simulink model "ASM_Traffic_new"  (R2024a)
settings: Solver=ode1  StartTime=SIM.tstart.v  StopTime=SIM.tend.v  FixedStep=SIM.StepSize.v  RelTol=1e-3
PostLoadFcn:
  | if any(exist('dsrtsu_mdlpostloadfcn', 'file') ~= 0), dsrtsu_mdlpostloadfcn('Execute', bdroot); end
  | try, asm_mdl_postloadfcn(bdroot, 'UpdateModel', 3600); catch, disp(lasterr); end,
InitFcn:
  | , if any(exist('rtifpga_mdlclblib', 'file') ~= 0), rtifpga_mdlclblib('Init', bdroot); end,
  | , if any(exist('dsmpb_private', 'file') ~= 0), dsmpb_private('dsmpb_mdlclblib', 'Init', bdroot); end,
undefined symbols (not defined in the file): _to_, a0b2, ASM_BrakeHydraulics_DemoSystems, ASM_VehicleDynamics_DemoSystems, b98103fe8ad365046cd0, BrakeCircuit, CPT, Crankshaft, DiscIntNeverNeededParam, dsmsi, FinalDriveAssembly, MDL, ModeSignals, Pos_BrakePedal_Maneuver, rad, RefSignals, s_to_rpm, SIM, SoftECU, Suspension, Tire, Transmission
libraries: ASM_Traffic_lib x135, simulink x100, ASM_Utils_lib x77, ASM_VehicleDynamics_lib x70, ASM_Environment_lib x22, dsmpblib x20, dsmsilib x15, MDLD_Utils_lib x10, ASM_BrakeHydraulics_lib x3
(part 61 of 63)

== system ASM_Traffic_new/Environment/GroundTruth/UserInterface/PAR_Plant/Fellow_Vehicles/Lightstates_Fellow25/Indicator_State[]/ASM_OSI_Mapping ==
  Fellow_TurnLights[] : Inport
  Table_ASM_To_OSI : Lookup_n-D  NumberOfTableDimensions=1  BreakpointsForDimension1=[0,1,2,3]  Table=[2,3,4,5]  InterpMethod=Nearest  InternalRulePriority=Speed  RndMeth=Simplest
  Indicator_State[] : Outport  VectorParamsAs1DForOutWhenUnconnected=off
  wires:
  Table_ASM_To_OSI/1 -> Indicator_State[]/1
  Fellow_TurnLights[]/1 -> Table_ASM_To_OSI/1

== system ASM_Traffic_new/Environment/GroundTruth/UserInterface/PAR_Plant/Fellow_Vehicles/Lightstates_Fellow26/Indicator_State[]/ASM_OSI_Mapping ==
  Fellow_TurnLights[] : Inport
  Table_ASM_To_OSI : Lookup_n-D  NumberOfTableDimensions=1  BreakpointsForDimension1=[0,1,2,3]  Table=[2,3,4,5]  InterpMethod=Nearest  InternalRulePriority=Speed  RndMeth=Simplest
  Indicator_State[] : Outport  VectorParamsAs1DForOutWhenUnconnected=off
  wires:
  Fellow_TurnLights[]/1 -> Table_ASM_To_OSI/1
  Table_ASM_To_OSI/1 -> Indicator_State[]/1

== system ASM_Traffic_new/Environment/GroundTruth/UserInterface/PAR_Plant/Fellow_Vehicles/Lightstates_Fellow27/Indicator_State[]/ASM_OSI_Mapping ==
  Fellow_TurnLights[] : Inport
  Table_ASM_To_OSI : Lookup_n-D  NumberOfTableDimensions=1  BreakpointsForDimension1=[0,1,2,3]  Table=[2,3,4,5]  InterpMethod=Nearest  InternalRulePriority=Speed  RndMeth=Simplest
  Indicator_State[] : Outport  VectorParamsAs1DForOutWhenUnconnected=off
  wires:
  Table_ASM_To_OSI/1 -> Indicator_State[]/1
  Fellow_TurnLights[]/1 -> Table_ASM_To_OSI/1

== system ASM_Traffic_new/Environment/GroundTruth/UserInterface/PAR_Plant/Fellow_Vehicles/Lightstates_Fellow28/Indicator_State[]/ASM_OSI_Mapping ==
  Fellow_TurnLights[] : Inport
  Table_ASM_To_OSI : Lookup_n-D  NumberOfTableDimensions=1  BreakpointsForDimension1=[0,1,2,3]  Table=[2,3,4,5]  InterpMethod=Nearest  InternalRulePriority=Speed  RndMeth=Simplest
  Indicator_State[] : Outport  VectorParamsAs1DForOutWhenUnconnected=off
  wires:
  Fellow_TurnLights[]/1 -> Table_ASM_To_OSI/1
  Table_ASM_To_OSI/1 -> Indicator_State[]/1

== system ASM_Traffic_new/Environment/GroundTruth/UserInterface/PAR_Plant/Fellow_Vehicles/Lightstates_Fellow29/Indicator_State[]/ASM_OSI_Mapping ==
  Fellow_TurnLights[] : Inport
  Table_ASM_To_OSI : Lookup_n-D  NumberOfTableDimensions=1  BreakpointsForDimension1=[0,1,2,3]  Table=[2,3,4,5]  InterpMethod=Nearest  InternalRulePriority=Speed  RndMeth=Simplest
  Indicator_State[] : Outport  VectorParamsAs1DForOutWhenUnconnected=off
  wires:
  Table_ASM_To_OSI/1 -> Indicator_State[]/1
  Fellow_TurnLights[]/1 -> Table_ASM_To_OSI/1

== system ASM_Traffic_new/Environment/GroundTruth/UserInterface/PAR_Plant/Fellow_Vehicles/Lightstates_Fellow3/Indicator_State[]/ASM_OSI_Mapping ==
  Fellow_TurnLights[] : Inport
  Table_ASM_To_OSI : Lookup_n-D  NumberOfTableDimensions=1  BreakpointsForDimension1=[0,1,2,3]  Table=[2,3,4,5]  InterpMethod=Nearest  InternalRulePriority=Speed  RndMeth=Simplest
  Indicator_State[] : Outport  VectorParamsAs1DForOutWhenUnconnected=off
  wires:
  Table_ASM_To_OSI/1 -> Indicator_State[]/1
  Fellow_TurnLights[]/1 -> Table_ASM_To_OSI/1

== system ASM_Traffic_new/Environment/GroundTruth/UserInterface/PAR_Plant/Fellow_Vehicles/Lightstates_Fellow30/Indicator_State[]/ASM_OSI_Mapping ==
  Fellow_TurnLights[] : Inport
  Table_ASM_To_OSI : Lookup_n-D  NumberOfTableDimensions=1  BreakpointsForDimension1=[0,1,2,3]  Table=[2,3,4,5]  InterpMethod=Nearest  InternalRulePriority=Speed  RndMeth=Simplest
  Indicator_State[] : Outport  VectorParamsAs1DForOutWhenUnconnected=off
  wires:
  Fellow_TurnLights[]/1 -> Table_ASM_To_OSI/1
  Table_ASM_To_OSI/1 -> Indicator_State[]/1

== system ASM_Traffic_new/Environment/GroundTruth/UserInterface/PAR_Plant/Fellow_Vehicles/Lightstates_Fellow4/Indicator_State[]/ASM_OSI_Mapping ==
  Fellow_TurnLights[] : Inport
  Table_ASM_To_OSI : Lookup_n-D  NumberOfTableDimensions=1  BreakpointsForDimension1=[0,1,2,3]  Table=[2,3,4,5]  InterpMethod=Nearest  InternalRulePriority=Speed  RndMeth=Simplest
  Indicator_State[] : Outport  VectorParamsAs1DForOutWhenUnconnected=off
  wires:
  Fellow_TurnLights[]/1 -> Table_ASM_To_OSI/1
  Table_ASM_To_OSI/1 -> Indicator_State[]/1

== system ASM_Traffic_new/Environment/GroundTruth/UserInterface/PAR_Plant/Fellow_Vehicles/Lightstates_Fellow5/Indicator_State[]/ASM_OSI_Mapping ==
  Fellow_TurnLights[] : Inport
  Table_ASM_To_OSI : Lookup_n-D  NumberOfTableDimensions=1  BreakpointsForDimension1=[0,1,2,3]  Table=[2,3,4,5]  InterpMethod=Nearest  InternalRulePriority=Speed  RndMeth=Simplest
  Indicator_State[] : Outport  VectorParamsAs1DForOutWhenUnconnected=off
  wires:
  Table_ASM_To_OSI/1 -> Indicator_State[]/1
  Fellow_TurnLights[]/1 -> Table_ASM_To_OSI/1

== system ASM_Traffic_new/Environment/GroundTruth/UserInterface/PAR_Plant/Fellow_Vehicles/Lightstates_Fellow6/Indicator_State[]/ASM_OSI_Mapping ==
  Fellow_TurnLights[] : Inport
  Table_ASM_To_OSI : Lookup_n-D  NumberOfTableDimensions=1  BreakpointsForDimension1=[0,1,2,3]  Table=[2,3,4,5]  InterpMethod=Nearest  InternalRulePriority=Speed  RndMeth=Simplest
  Indicator_State[] : Outport  VectorParamsAs1DForOutWhenUnconnected=off
  wires:
  Fellow_TurnLights[]/1 -> Table_ASM_To_OSI/1
  Table_ASM_To_OSI/1 -> Indicator_State[]/1

== system ASM_Traffic_new/Environment/GroundTruth/UserInterface/PAR_Plant/Fellow_Vehicles/Lightstates_Fellow7/Indicator_State[]/ASM_OSI_Mapping ==
  Fellow_TurnLights[] : Inport
  Table_ASM_To_OSI : Lookup_n-D  NumberOfTableDimensions=1  BreakpointsForDimension1=[0,1,2,3]  Table=[2,3,4,5]  InterpMethod=Nearest  InternalRulePriority=Speed  RndMeth=Simplest
  Indicator_State[] : Outport  VectorParamsAs1DForOutWhenUnconnected=off
  wires:
  Table_ASM_To_OSI/1 -> Indicator_State[]/1
  Fellow_TurnLights[]/1 -> Table_ASM_To_OSI/1

== system ASM_Traffic_new/Environment/GroundTruth/UserInterface/PAR_Plant/Fellow_Vehicles/Lightstates_Fellow8/Indicator_State[]/ASM_OSI_Mapping ==
  Fellow_TurnLights[] : Inport
  Table_ASM_To_OSI : Lookup_n-D  NumberOfTableDimensions=1  BreakpointsForDimension1=[0,1,2,3]  Table=[2,3,4,5]  InterpMethod=Nearest  InternalRulePriority=Speed  RndMeth=Simplest
  Indicator_State[] : Outport  VectorParamsAs1DForOutWhenUnconnected=off
  wires:
  Fellow_TurnLights[]/1 -> Table_ASM_To_OSI/1
  Table_ASM_To_OSI/1 -> Indicator_State[]/1

== system ASM_Traffic_new/Environment/GroundTruth/UserInterface/PAR_Plant/Fellow_Vehicles/Lightstates_Fellow9/Indicator_State[]/ASM_OSI_Mapping ==
  Fellow_TurnLights[] : Inport
  Table_ASM_To_OSI : Lookup_n-D  NumberOfTableDimensions=1  BreakpointsForDimension1=[0,1,2,3]  Table=[2,3,4,5]  InterpMethod=Nearest  InternalRulePriority=Speed  RndMeth=Simplest
  Indicator_State[] : Outport  VectorParamsAs1DForOutWhenUnconnected=off
  wires:
  Table_ASM_To_OSI/1 -> Indicator_State[]/1
  Fellow_TurnLights[]/1 -> Table_ASM_To_OSI/1

== system ASM_Traffic_new/Environment/Sensors/PlantModel/Object_Sensor_2D/ObjectData/Sensor1/Object_Custom_Values/Vectorize_Signals ==
  SensorOutput1 : Inport
  SensorOutput2 : Inport  Port=2
  SensorOutput3 : Inport  Port=3
  Bus Creator : BusCreator  Inputs=2
  Bus Selector : BusSelector  OutputSignals=SensorOutput.Object1.Object_Valid[0|1],SensorOutput.Object2.Object_Valid[0|1],SensorOutput.Object3.Object_Valid[0|1],SensorOutput.Object4.Object_Valid[0|1],SensorOutput.Object5.Object_Valid[0|1]
  Bus Selector1 : BusSelector  OutputSignals=SensorOutput.Object1.Object_Valid[0|1],SensorOutput.Object2.Object_Valid[0|1],SensorOutput.Object3.Object_Valid[0|1],SensorOutput.Object4.Object_Valid[0|1],SensorOutput.Object5.Object_Valid[0|1]
  Bus Selector2 : BusSelector  OutputSignals=SensorOutput.Object1.Object_Valid[0|1],SensorOutput.Object2.Object_Valid[0|1],SensorOutput.Object3.Object_Valid[0|1],SensorOutput.Object4.Object_Valid[0|1],SensorOutput.Object5.Object_Valid[0|1]
  Bus Selector3 : BusSelector  OutputSignals=SensorOutput.Object1.CustomValues[],SensorOutput.Object2.CustomValues[],SensorOutput.Object3.CustomValues[],SensorOutput.Object4.CustomValues[],SensorOutput.Object5.CustomValues[]
  Bus Selector4 : BusSelector  OutputSignals=SensorOutput.Object1.CustomValues[],SensorOutput.Object2.CustomValues[],SensorOutput.Object3.CustomValues[],SensorOutput.Object4.CustomValues[],SensorOutput.Object5.CustomValues[]
  Bus Selector5 : BusSelector  OutputSignals=SensorOutput.Object1.CustomValues[],SensorOutput.Object2.CustomValues[],SensorOutput.Object3.CustomValues[],SensorOutput.Object4.CustomValues[],SensorOutput.Object5.CustomValues[]
  Mux : Mux  Inputs=15
  Mux1 : Mux  Inputs=15
  Vectorized_Custom_Values : Outport  VectorParamsAs1DForOutWhenUnconnected=off
  wires:
  Bus Creator/1 -> Vectorized_Custom_Values/1
  Bus Selector5/5 -> Mux1/15  "<CustomValues[]>"
  Bus Selector5/4 -> Mux1/14  "<CustomValues[]>"
  Bus Selector5/3 -> Mux1/13  "<CustomValues[]>"
  Bus Selector5/2 -> Mux1/12  "<CustomValues[]>"
  Bus Selector5/1 -> Mux1/11  "<CustomValues[]>"
  Bus Selector4/5 -> Mux1/10  "<CustomValues[]>"
  Bus Selector4/4 -> Mux1/9  "<CustomValues[]>"
  Bus Selector4/3 -> Mux1/8  "<CustomValues[]>"
  Bus Selector4/2 -> Mux1/7  "<CustomValues[]>"
  Bus Selector4/1 -> Mux1/6  "<CustomValues[]>"
  Bus Selector3/5 -> Mux1/5  "<CustomValues[]>"
  Bus Selector3/4 -> Mux1/4  "<CustomValues[]>"
  Bus Selector3/3 -> Mux1/3  "<CustomValues[]>"
  Bus Selector3/2 -> Mux1/2  "<CustomValues[]>"
  Bus Selector3/1 -> Mux1/1  "<CustomValues[]>"
  Bus Selector2/5 -> Mux/15  "<Object_Valid[0|1]>"
  Bus Selector2/4 -> Mux/14  "<Object_Valid[0|1]>"
  Bus Selector2/3 -> Mux/13  "<Object_Valid[0|1]>"
  Bus Selector2/2 -> Mux/12  "<Object_Valid[0|1]>"
  Bus Selector2/1 -> Mux/11  "<Object_Valid[0|1]>"
  Bus Selector1/5 -> Mux/10  "<Object_Valid[0|1]>"
  Bus Selector1/4 -> Mux/9  "<Object_Valid[0|1]>"
  Bus Selector1/3 -> Mux/8  "<Object_Valid[0|1]>"
  Bus Selector1/2 -> Mux/7  "<Object_Valid[0|1]>"
  Bus Selector1/1 -> Mux/6  "<Object_Valid[0|1]>"
  Mux1/1 -> Bus Creator/2  "CustomValues[]"
  Mux/1 -> Bus Creator/1  "Object_Valid[0|1]"
  SensorOutput3/1 -> Bus Selector2/1, Bus Selector5/1
  SensorOutput2/1 -> Bus Selector1/1, Bus Selector4/1
  Bus Selector/1 -> Mux/1  "<Object_Valid[0|1]>"
  Bus Selector/2 -> Mux/2  "<Object_Valid[0|1]>"
  Bus Selector/3 -> Mux/3  "<Object_Valid[0|1]>"
  Bus Selector/4 -> Mux/4  "<Object_Valid[0|1]>"
  Bus Selector/5 -> Mux/5  "<Object_Valid[0|1]>"
  SensorOutput1/1 -> Bus Selector3/1, Bus Selector/1

== system ASM_Traffic_new/Environment/Sensors/PlantModel/Object_Sensor_2D/ObjectData/Sensor2/Object_Custom_Values/Vectorize_Signals ==
  SensorOutput1 : Inport
  SensorOutput2 : Inport  Port=2
  SensorOutput3 : Inport  Port=3
  Bus Creator : BusCreator  Inputs=2
  Bus Selector : BusSelector  OutputSignals=SensorOutput.Object1.Object_Valid[0|1],SensorOutput.Object2.Object_Valid[0|1],SensorOutput.Object3.Object_Valid[0|1],SensorOutput.Object4.Object_Valid[0|1],SensorOutput.Object5.Object_Valid[0|1]
  Bus Selector1 : BusSelector  OutputSignals=SensorOutput.Object1.Object_Valid[0|1],SensorOutput.Object2.Object_Valid[0|1],SensorOutput.Object3.Object_Valid[0|1],SensorOutput.Object4.Object_Valid[0|1],SensorOutput.Object5.Object_Valid[0|1]
  Bus Selector2 : BusSelector  OutputSignals=SensorOutput.Object1.Object_Valid[0|1],SensorOutput.Object2.Object_Valid[0|1],SensorOutput.Object3.Object_Valid[0|1],SensorOutput.Object4.Object_Valid[0|1],SensorOutput.Object5.Object_Valid[0|1]
  Bus Selector3 : BusSelector  OutputSignals=SensorOutput.Object1.CustomValues[],SensorOutput.Object2.CustomValues[],SensorOutput.Object3.CustomValues[],SensorOutput.Object4.CustomValues[],SensorOutput.Object5.CustomValues[]
  Bus Selector4 : BusSelector  OutputSignals=SensorOutput.Object1.CustomValues[],SensorOutput.Object2.CustomValues[],SensorOutput.Object3.CustomValues[],SensorOutput.Object4.CustomValues[],SensorOutput.Object5.CustomValues[]
  Bus Selector5 : BusSelector  OutputSignals=SensorOutput.Object1.CustomValues[],SensorOutput.Object2.CustomValues[],SensorOutput.Object3.CustomValues[],SensorOutput.Object4.CustomValues[],SensorOutput.Object5.CustomValues[]
  Mux : Mux  Inputs=15
  Mux1 : Mux  Inputs=15
  Vectorized_Custom_Values : Outport  VectorParamsAs1DForOutWhenUnconnected=off
  wires:
  SensorOutput1/1 -> Bus Selector/1, Bus Selector3/1
  Bus Selector/5 -> Mux/5  "<Object_Valid[0|1]>"
  Bus Selector/4 -> Mux/4  "<Object_Valid[0|1]>"
  Bus Selector/3 -> Mux/3  "<Object_Valid[0|1]>"
  Bus Selector/2 -> Mux/2  "<Object_Valid[0|1]>"
  Bus Selector/1 -> Mux/1  "<Object_Valid[0|1]>"
  SensorOutput2/1 -> Bus Selector4/1, Bus Selector1/1
  SensorOutput3/1 -> Bus Selector5/1, Bus Selector2/1
  Mux/1 -> Bus Creator/1  "Object_Valid[0|1]"
  Mux1/1 -> Bus Creator/2  "CustomValues[]"
  Bus Selector1/1 -> Mux/6  "<Object_Valid[0|1]>"
  Bus Selector1/2 -> Mux/7  "<Object_Valid[0|1]>"
  Bus Selector1/3 -> Mux/8  "<Object_Valid[0|1]>"
  Bus Selector1/4 -> Mux/9  "<Object_Valid[0|1]>"
  Bus Selector1/5 -> Mux/10  "<Object_Valid[0|1]>"
  Bus Selector2/1 -> Mux/11  "<Object_Valid[0|1]>"
  Bus Selector2/2 -> Mux/12  "<Object_Valid[0|1]>"
  Bus Selector2/3 -> Mux/13  "<Object_Valid[0|1]>"
  Bus Selector2/4 -> Mux/14  "<Object_Valid[0|1]>"
  Bus Selector2/5 -> Mux/15  "<Object_Valid[0|1]>"
  Bus Selector3/1 -> Mux1/1  "<CustomValues[]>"
  Bus Selector3/2 -> Mux1/2  "<CustomValues[]>"
  Bus Selector3/3 -> Mux1/3  "<CustomValues[]>"
  Bus Selector3/4 -> Mux1/4  "<CustomValues[]>"
  Bus Selector3/5 -> Mux1/5  "<CustomValues[]>"
  Bus Selector4/1 -> Mux1/6  "<CustomValues[]>"
  Bus Selector4/2 -> Mux1/7  "<CustomValues[]>"
  Bus Selector4/3 -> Mux1/8  "<CustomValues[]>"
  Bus Selector4/4 -> Mux1/9  "<CustomValues[]>"
  Bus Selector4/5 -> Mux1/10  "<CustomValues[]>"
  Bus Selector5/1 -> Mux1/11  "<CustomValues[]>"
  Bus Selector5/2 -> Mux1/12  "<CustomValues[]>"
  Bus Selector5/3 -> Mux1/13  "<CustomValues[]>"
  Bus Selector5/4 -> Mux1/14  "<CustomValues[]>"
  Bus Selector5/5 -> Mux1/15  "<CustomValues[]>"
  Bus Creator/1 -> Vectorized_Custom_Values/1

== system ASM_Traffic_new/Environment/Sensors/PlantModel/Object_Sensor_2D/ObjectData/Sensor3/Object_Custom_Values/Vectorize_Signals ==
  SensorOutput1 : Inport
  SensorOutput2 : Inport  Port=2
  SensorOutput3 : Inport  Port=3
  Bus Creator : BusCreator  Inputs=2
  Bus Selector : BusSelector  OutputSignals=SensorOutput.Object1.Object_Valid[0|1],SensorOutput.Object2.Object_Valid[0|1],SensorOutput.Object3.Object_Valid[0|1],SensorOutput.Object4.Object_Valid[0|1],SensorOutput.Object5.Object_Valid[0|1]
  Bus Selector1 : BusSelector  OutputSignals=SensorOutput.Object1.Object_Valid[0|1],SensorOutput.Object2.Object_Valid[0|1],SensorOutput.Object3.Object_Valid[0|1],SensorOutput.Object4.Object_Valid[0|1],SensorOutput.Object5.Object_Valid[0|1]
  Bus Selector2 : BusSelector  OutputSignals=SensorOutput.Object1.Object_Valid[0|1],SensorOutput.Object2.Object_Valid[0|1],SensorOutput.Object3.Object_Valid[0|1],SensorOutput.Object4.Object_Valid[0|1],SensorOutput.Object5.Object_Valid[0|1]
  Bus Selector3 : BusSelector  OutputSignals=SensorOutput.Object1.CustomValues[],SensorOutput.Object2.CustomValues[],SensorOutput.Object3.CustomValues[],SensorOutput.Object4.CustomValues[],SensorOutput.Object5.CustomValues[]
  Bus Selector4 : BusSelector  OutputSignals=SensorOutput.Object1.CustomValues[],SensorOutput.Object2.CustomValues[],SensorOutput.Object3.CustomValues[],SensorOutput.Object4.CustomValues[],SensorOutput.Object5.CustomValues[]
  Bus Selector5 : BusSelector  OutputSignals=SensorOutput.Object1.CustomValues[],SensorOutput.Object2.CustomValues[],SensorOutput.Object3.CustomValues[],SensorOutput.Object4.CustomValues[],SensorOutput.Object5.CustomValues[]
  Mux : Mux  Inputs=15
  Mux1 : Mux  Inputs=15
  Vectorized_Custom_Values : Outport  VectorParamsAs1DForOutWhenUnconnected=off
  wires:
  Bus Creator/1 -> Vectorized_Custom_Values/1
  Bus Selector5/5 -> Mux1/15  "<CustomValues[]>"
  Bus Selector5/4 -> Mux1/14  "<CustomValues[]>"
  Bus Selector5/3 -> Mux1/13  "<CustomValues[]>"
  Bus Selector5/2 -> Mux1/12  "<CustomValues[]>"
  Bus Selector5/1 -> Mux1/11  "<CustomValues[]>"
  Bus Selector4/5 -> Mux1/10  "<CustomValues[]>"
  Bus Selector4/4 -> Mux1/9  "<CustomValues[]>"
  Bus Selector4/3 -> Mux1/8  "<CustomValues[]>"
  Bus Selector4/2 -> Mux1/7  "<CustomValues[]>"
  Bus Selector4/1 -> Mux1/6  "<CustomValues[]>"
  Bus Selector3/5 -> Mux1/5  "<CustomValues[]>"
  Bus Selector3/4 -> Mux1/4  "<CustomValues[]>"
  Bus Selector3/3 -> Mux1/3  "<CustomValues[]>"
  Bus Selector3/2 -> Mux1/2  "<CustomValues[]>"
  Bus Selector3/1 -> Mux1/1  "<CustomValues[]>"
  Bus Selector2/5 -> Mux/15  "<Object_Valid[0|1]>"
  Bus Selector2/4 -> Mux/14  "<Object_Valid[0|1]>"
  Bus Selector2/3 -> Mux/13  "<Object_Valid[0|1]>"
  Bus Selector2/2 -> Mux/12  "<Object_Valid[0|1]>"
  Bus Selector2/1 -> Mux/11  "<Object_Valid[0|1]>"
  Bus Selector1/5 -> Mux/10  "<Object_Valid[0|1]>"
  Bus Selector1/4 -> Mux/9  "<Object_Valid[0|1]>"
  Bus Selector1/3 -> Mux/8  "<Object_Valid[0|1]>"
  Bus Selector1/2 -> Mux/7  "<Object_Valid[0|1]>"
  Bus Selector1/1 -> Mux/6  "<Object_Valid[0|1]>"
  Mux1/1 -> Bus Creator/2  "CustomValues[]"
  Mux/1 -> Bus Creator/1  "Object_Valid[0|1]"
  SensorOutput3/1 -> Bus Selector2/1, Bus Selector5/1
  SensorOutput2/1 -> Bus Selector1/1, Bus Selector4/1
  Bus Selector/1 -> Mux/1  "<Object_Valid[0|1]>"
  Bus Selector/2 -> Mux/2  "<Object_Valid[0|1]>"
  Bus Selector/3 -> Mux/3  "<Object_Valid[0|1]>"
  Bus Selector/4 -> Mux/4  "<Object_Valid[0|1]>"
  Bus Selector/5 -> Mux/5  "<Object_Valid[0|1]>"
  SensorOutput1/1 -> Bus Selector3/1, Bus Selector/1

== system ASM_Traffic_new/Environment/Sensors/PlantModel/Object_Sensor_2D/ObjectData/Sensor4/Object_Custom_Values/Vectorize_Signals ==
  SensorOutput1 : Inport
  SensorOutput2 : Inport  Port=2
  SensorOutput3 : Inport  Port=3
  Bus Creator : BusCreator  Inputs=2
  Bus Selector : BusSelector  OutputSignals=SensorOutput.Object1.Object_Valid[0|1],SensorOutput.Object2.Object_Valid[0|1],SensorOutput.Object3.Object_Valid[0|1],SensorOutput.Object4.Object_Valid[0|1],SensorOutput.Object5.Object_Valid[0|1]
  Bus Selector1 : BusSelector  OutputSignals=SensorOutput.Object1.Object_Valid[0|1],SensorOutput.Object2.Object_Valid[0|1],SensorOutput.Object3.Object_Valid[0|1],SensorOutput.Object4.Object_Valid[0|1],SensorOutput.Object5.Object_Valid[0|1]
  Bus Selector2 : BusSelector  OutputSignals=SensorOutput.Object1.Object_Valid[0|1],SensorOutput.Object2.Object_Valid[0|1],SensorOutput.Object3.Object_Valid[0|1],SensorOutput.Object4.Object_Valid[0|1],SensorOutput.Object5.Object_Valid[0|1]
  Bus Selector3 : BusSelector  OutputSignals=SensorOutput.Object1.CustomValues[],SensorOutput.Object2.CustomValues[],SensorOutput.Object3.CustomValues[],SensorOutput.Object4.CustomValues[],SensorOutput.Object5.CustomValues[]
  Bus Selector4 : BusSelector  OutputSignals=SensorOutput.Object1.CustomValues[],SensorOutput.Object2.CustomValues[],SensorOutput.Object3.CustomValues[],SensorOutput.Object4.CustomValues[],SensorOutput.Object5.CustomValues[]
  Bus Selector5 : BusSelector  OutputSignals=SensorOutput.Object1.CustomValues[],SensorOutput.Object2.CustomValues[],SensorOutput.Object3.CustomValues[],SensorOutput.Object4.CustomValues[],SensorOutput.Object5.CustomValues[]
  Mux : Mux  Inputs=15
  Mux1 : Mux  Inputs=15
  Vectorized_Custom_Values : Outport  VectorParamsAs1DForOutWhenUnconnected=off
  wires:
  Bus Creator/1 -> Vectorized_Custom_Values/1
  Bus Selector5/5 -> Mux1/15  "<CustomValues[]>"
  Bus Selector5/4 -> Mux1/14  "<CustomValues[]>"
  Bus Selector5/3 -> Mux1/13  "<CustomValues[]>"
  Bus Selector5/2 -> Mux1/12  "<CustomValues[]>"
  Bus Selector5/1 -> Mux1/11  "<CustomValues[]>"
  Bus Selector4/5 -> Mux1/10  "<CustomValues[]>"
  Bus Selector4/4 -> Mux1/9  "<CustomValues[]>"
  Bus Selector4/3 -> Mux1/8  "<CustomValues[]>"
  Bus Selector4/2 -> Mux1/7  "<CustomValues[]>"
  Bus Selector4/1 -> Mux1/6  "<CustomValues[]>"
  Bus Selector3/5 -> Mux1/5  "<CustomValues[]>"
  Bus Selector3/4 -> Mux1/4  "<CustomValues[]>"
  Bus Selector3/3 -> Mux1/3  "<CustomValues[]>"
  Bus Selector3/2 -> Mux1/2  "<CustomValues[]>"
  Bus Selector3/1 -> Mux1/1  "<CustomValues[]>"
  Bus Selector2/5 -> Mux/15  "<Object_Valid[0|1]>"
  Bus Selector2/4 -> Mux/14  "<Object_Valid[0|1]>"
  Bus Selector2/3 -> Mux/13  "<Object_Valid[0|1]>"
  Bus Selector2/2 -> Mux/12  "<Object_Valid[0|1]>"
  Bus Selector2/1 -> Mux/11  "<Object_Valid[0|1]>"
  Bus Selector1/5 -> Mux/10  "<Object_Valid[0|1]>"
  Bus Selector1/4 -> Mux/9  "<Object_Valid[0|1]>"
  Bus Selector1/3 -> Mux/8  "<Object_Valid[0|1]>"
  Bus Selector1/2 -> Mux/7  "<Object_Valid[0|1]>"
  Bus Selector1/1 -> Mux/6  "<Object_Valid[0|1]>"
  Mux1/1 -> Bus Creator/2  "CustomValues[]"
  Mux/1 -> Bus Creator/1  "Object_Valid[0|1]"
  SensorOutput3/1 -> Bus Selector2/1, Bus Selector5/1
  SensorOutput2/1 -> Bus Selector1/1, Bus Selector4/1
  Bus Selector/1 -> Mux/1  "<Object_Valid[0|1]>"
  Bus Selector/2 -> Mux/2  "<Object_Valid[0|1]>"
  Bus Selector/3 -> Mux/3  "<Object_Valid[0|1]>"
  Bus Selector/4 -> Mux/4  "<Object_Valid[0|1]>"
  Bus Selector/5 -> Mux/5  "<Object_Valid[0|1]>"
  SensorOutput1/1 -> Bus Selector3/1, Bus Selector/1

== system ASM_Traffic_new/Environment/Sensors/PlantModel/Object_Sensor_2D/ObjectData/Sensor5/Object_Custom_Values/Vectorize_Signals ==
  SensorOutput1 : Inport
  SensorOutput2 : Inport  Port=2
  SensorOutput3 : Inport  Port=3
  Bus Creator : BusCreator  Inputs=2
  Bus Selector : BusSelector  OutputSignals=SensorOutput.Object1.Object_Valid[0|1],SensorOutput.Object2.Object_Valid[0|1],SensorOutput.Object3.Object_Valid[0|1],SensorOutput.Object4.Object_Valid[0|1],SensorOutput.Object5.Object_Valid[0|1]
  Bus Selector1 : BusSelector  OutputSignals=SensorOutput.Object1.Object_Valid[0|1],SensorOutput.Object2.Object_Valid[0|1],SensorOutput.Object3.Object_Valid[0|1],SensorOutput.Object4.Object_Valid[0|1],SensorOutput.Object5.Object_Valid[0|1]
  Bus Selector2 : BusSelector  OutputSignals=SensorOutput.Object1.Object_Valid[0|1],SensorOutput.Object2.Object_Valid[0|1],SensorOutput.Object3.Object_Valid[0|1],SensorOutput.Object4.Object_Valid[0|1],SensorOutput.Object5.Object_Valid[0|1]
  Bus Selector3 : BusSelector  OutputSignals=SensorOutput.Object1.CustomValues[],SensorOutput.Object2.CustomValues[],SensorOutput.Object3.CustomValues[],SensorOutput.Object4.CustomValues[],SensorOutput.Object5.CustomValues[]
  Bus Selector4 : BusSelector  OutputSignals=SensorOutput.Object1.CustomValues[],SensorOutput.Object2.CustomValues[],SensorOutput.Object3.CustomValues[],SensorOutput.Object4.CustomValues[],SensorOutput.Object5.CustomValues[]
  Bus Selector5 : BusSelector  OutputSignals=SensorOutput.Object1.CustomValues[],SensorOutput.Object2.CustomValues[],SensorOutput.Object3.CustomValues[],SensorOutput.Object4.CustomValues[],SensorOutput.Object5.CustomValues[]
  Mux : Mux  Inputs=15
  Mux1 : Mux  Inputs=15
  Vectorized_Custom_Values : Outport  VectorParamsAs1DForOutWhenUnconnected=off
  wires:
  SensorOutput1/1 -> Bus Selector/1, Bus Selector3/1
  Bus Selector/5 -> Mux/5  "<Object_Valid[0|1]>"
  Bus Selector/4 -> Mux/4  "<Object_Valid[0|1]>"
  Bus Selector/3 -> Mux/3  "<Object_Valid[0|1]>"
  Bus Selector/2 -> Mux/2  "<Object_Valid[0|1]>"
  Bus Selector/1 -> Mux/1  "<Object_Valid[0|1]>"
  SensorOutput2/1 -> Bus Selector4/1, Bus Selector1/1
  SensorOutput3/1 -> Bus Selector5/1, Bus Selector2/1
  Mux/1 -> Bus Creator/1  "Object_Valid[0|1]"
  Mux1/1 -> Bus Creator/2  "CustomValues[]"
  Bus Selector1/1 -> Mux/6  "<Object_Valid[0|1]>"
  Bus Selector1/2 -> Mux/7  "<Object_Valid[0|1]>"
  Bus Selector1/3 -> Mux/8  "<Object_Valid[0|1]>"
  Bus Selector1/4 -> Mux/9  "<Object_Valid[0|1]>"
  Bus Selector1/5 -> Mux/10  "<Object_Valid[0|1]>"
  Bus Selector2/1 -> Mux/11  "<Object_Valid[0|1]>"
  Bus Selector2/2 -> Mux/12  "<Object_Valid[0|1]>"
  Bus Selector2/3 -> Mux/13  "<Object_Valid[0|1]>"
  Bus Selector2/4 -> Mux/14  "<Object_Valid[0|1]>"
  Bus Selector2/5 -> Mux/15  "<Object_Valid[0|1]>"
  Bus Selector3/1 -> Mux1/1  "<CustomValues[]>"
  Bus Selector3/2 -> Mux1/2  "<CustomValues[]>"
  Bus Selector3/3 -> Mux1/3  "<CustomValues[]>"
  Bus Selector3/4 -> Mux1/4  "<CustomValues[]>"
  Bus Selector3/5 -> Mux1/5  "<CustomValues[]>"
  Bus Selector4/1 -> Mux1/6  "<CustomValues[]>"
  Bus Selector4/2 -> Mux1/7  "<CustomValues[]>"
  Bus Selector4/3 -> Mux1/8  "<CustomValues[]>"
  Bus Selector4/4 -> Mux1/9  "<CustomValues[]>"
  Bus Selector4/5 -> Mux1/10  "<CustomValues[]>"
  Bus Selector5/1 -> Mux1/11  "<CustomValues[]>"
  Bus Selector5/2 -> Mux1/12  "<CustomValues[]>"
  Bus Selector5/3 -> Mux1/13  "<CustomValues[]>"
  Bus Selector5/4 -> Mux1/14  "<CustomValues[]>"
  Bus Selector5/5 -> Mux1/15  "<CustomValues[]>"
  Bus Creator/1 -> Vectorized_Custom_Values/1

== system ASM_Traffic_new/Environment/Sensors/PlantModel/Object_Sensor_2D/ObjectData/Sensor6/Object_Custom_Values/Vectorize_Signals ==
  SensorOutput1 : Inport
  SensorOutput2 : Inport  Port=2
  SensorOutput3 : Inport  Port=3
  Bus Creator : BusCreator  Inputs=2
  Bus Selector : BusSelector  OutputSignals=SensorOutput.Object1.Object_Valid[0|1],SensorOutput.Object2.Object_Valid[0|1],SensorOutput.Object3.Object_Valid[0|1],SensorOutput.Object4.Object_Valid[0|1],SensorOutput.Object5.Object_Valid[0|1]
  Bus Selector1 : BusSelector  OutputSignals=SensorOutput.Object1.Object_Valid[0|1],SensorOutput.Object2.Object_Valid[0|1],SensorOutput.Object3.Object_Valid[0|1],SensorOutput.Object4.Object_Valid[0|1],SensorOutput.Object5.Object_Valid[0|1]
  Bus Selector2 : BusSelector  OutputSignals=SensorOutput.Object1.Object_Valid[0|1],SensorOutput.Object2.Object_Valid[0|1],SensorOutput.Object3.Object_Valid[0|1],SensorOutput.Object4.Object_Valid[0|1],SensorOutput.Object5.Object_Valid[0|1]
  Bus Selector3 : BusSelector  OutputSignals=SensorOutput.Object1.CustomValues[],SensorOutput.Object2.CustomValues[],SensorOutput.Object3.CustomValues[],SensorOutput.Object4.CustomValues[],SensorOutput.Object5.CustomValues[]
  Bus Selector4 : BusSelector  OutputSignals=SensorOutput.Object1.CustomValues[],SensorOutput.Object2.CustomValues[],SensorOutput.Object3.CustomValues[],SensorOutput.Object4.CustomValues[],SensorOutput.Object5.CustomValues[]
  Bus Selector5 : BusSelector  OutputSignals=SensorOutput.Object1.CustomValues[],SensorOutput.Object2.CustomValues[],SensorOutput.Object3.CustomValues[],SensorOutput.Object4.CustomValues[],SensorOutput.Object5.CustomValues[]
  Mux : Mux  Inputs=15
  Mux1 : Mux  Inputs=15
  Vectorized_Custom_Values : Outport  VectorParamsAs1DForOutWhenUnconnected=off
  wires:
  Bus Creator/1 -> Vectorized_Custom_Values/1
  Bus Selector5/5 -> Mux1/15  "<CustomValues[]>"
  Bus Selector5/4 -> Mux1/14  "<CustomValues[]>"
  Bus Selector5/3 -> Mux1/13  "<CustomValues[]>"
  Bus Selector5/2 -> Mux1/12  "<CustomValues[]>"
  Bus Selector5/1 -> Mux1/11  "<CustomValues[]>"
  Bus Selector4/5 -> Mux1/10  "<CustomValues[]>"
  Bus Selector4/4 -> Mux1/9  "<CustomValues[]>"
  Bus Selector4/3 -> Mux1/8  "<CustomValues[]>"
  Bus Selector4/2 -> Mux1/7  "<CustomValues[]>"
  Bus Selector4/1 -> Mux1/6  "<CustomValues[]>"
  Bus Selector3/5 -> Mux1/5  "<CustomValues[]>"
  Bus Selector3/4 -> Mux1/4  "<CustomValues[]>"
  Bus Selector3/3 -> Mux1/3  "<CustomValues[]>"
  Bus Selector3/2 -> Mux1/2  "<CustomValues[]>"
  Bus Selector3/1 -> Mux1/1  "<CustomValues[]>"
  Bus Selector2/5 -> Mux/15  "<Object_Valid[0|1]>"
  Bus Selector2/4 -> Mux/14  "<Object_Valid[0|1]>"
  Bus Selector2/3 -> Mux/13  "<Object_Valid[0|1]>"
  Bus Selector2/2 -> Mux/12  "<Object_Valid[0|1]>"
  Bus Selector2/1 -> Mux/11  "<Object_Valid[0|1]>"
  Bus Selector1/5 -> Mux/10  "<Object_Valid[0|1]>"
  Bus Selector1/4 -> Mux/9  "<Object_Valid[0|1]>"
  Bus Selector1/3 -> Mux/8  "<Object_Valid[0|1]>"
  Bus Selector1/2 -> Mux/7  "<Object_Valid[0|1]>"
  Bus Selector1/1 -> Mux/6  "<Object_Valid[0|1]>"
  Mux1/1 -> Bus Creator/2  "CustomValues[]"
  Mux/1 -> Bus Creator/1  "Object_Valid[0|1]"
  SensorOutput3/1 -> Bus Selector2/1, Bus Selector5/1
  SensorOutput2/1 -> Bus Selector1/1, Bus Selector4/1
  Bus Selector/1 -> Mux/1  "<Object_Valid[0|1]>"
  Bus Selector/2 -> Mux/2  "<Object_Valid[0|1]>"
  Bus Selector/3 -> Mux/3  "<Object_Valid[0|1]>"
  Bus Selector/4 -> Mux/4  "<Object_Valid[0|1]>"
  Bus Selector/5 -> Mux/5  "<Object_Valid[0|1]>"
  SensorOutput1/1 -> Bus Selector3/1, Bus Selector/1

== system ASM_Traffic_new/Environment/Sensors/PlantModel/Object_Sensor_2D/ObjectData/Sensor7/Object_Custom_Values/Vectorize_Signals ==
  SensorOutput1 : Inport
  SensorOutput2 : Inport  Port=2
  SensorOutput3 : Inport  Port=3
  Bus Creator : BusCreator  Inputs=2
  Bus Selector : BusSelector  OutputSignals=SensorOutput.Object1.Object_Valid[0|1],SensorOutput.Object2.Object_Valid[0|1],SensorOutput.Object3.Object_Valid[0|1],SensorOutput.Object4.Object_Valid[0|1],SensorOutput.Object5.Object_Valid[0|1]
  Bus Selector1 : BusSelector  OutputSignals=SensorOutput.Object1.Object_Valid[0|1],SensorOutput.Object2.Object_Valid[0|1],SensorOutput.Object3.Object_Valid[0|1],SensorOutput.Object4.Object_Valid[0|1],SensorOutput.Object5.Object_Valid[0|1]
  Bus Selector2 : BusSelector  OutputSignals=SensorOutput.Object1.Object_Valid[0|1],SensorOutput.Object2.Object_Valid[0|1],SensorOutput.Object3.Object_Valid[0|1],SensorOutput.Object4.Object_Valid[0|1],SensorOutput.Object5.Object_Valid[0|1]
  Bus Selector3 : BusSelector  OutputSignals=SensorOutput.Object1.CustomValues[],SensorOutput.Object2.CustomValues[],SensorOutput.Object3.CustomValues[],SensorOutput.Object4.CustomValues[],SensorOutput.Object5.CustomValues[]
  Bus Selector4 : BusSelector  OutputSignals=SensorOutput.Object1.CustomValues[],SensorOutput.Object2.CustomValues[],SensorOutput.Object3.CustomValues[],SensorOutput.Object4.CustomValues[],SensorOutput.Object5.CustomValues[]
  Bus Selector5 : BusSelector  OutputSignals=SensorOutput.Object1.CustomValues[],SensorOutput.Object2.CustomValues[],SensorOutput.Object3.CustomValues[],SensorOutput.Object4.CustomValues[],SensorOutput.Object5.CustomValues[]
  Mux : Mux  Inputs=15
  Mux1 : Mux  Inputs=15
  Vectorized_Custom_Values : Outport  VectorParamsAs1DForOutWhenUnconnected=off
  wires:
  SensorOutput1/1 -> Bus Selector/1, Bus Selector3/1
  Bus Selector/5 -> Mux/5  "<Object_Valid[0|1]>"
  Bus Selector/4 -> Mux/4  "<Object_Valid[0|1]>"
  Bus Selector/3 -> Mux/3  "<Object_Valid[0|1]>"
  Bus Selector/2 -> Mux/2  "<Object_Valid[0|1]>"
  Bus Selector/1 -> Mux/1  "<Object_Valid[0|1]>"
  SensorOutput2/1 -> Bus Selector4/1, Bus Selector1/1
  SensorOutput3/1 -> Bus Selector5/1, Bus Selector2/1
  Mux/1 -> Bus Creator/1  "Object_Valid[0|1]"
  Mux1/1 -> Bus Creator/2  "CustomValues[]"
  Bus Selector1/1 -> Mux/6  "<Object_Valid[0|1]>"
  Bus Selector1/2 -> Mux/7  "<Object_Valid[0|1]>"
  Bus Selector1/3 -> Mux/8  "<Object_Valid[0|1]>"
  Bus Selector1/4 -> Mux/9  "<Object_Valid[0|1]>"
  Bus Selector1/5 -> Mux/10  "<Object_Valid[0|1]>"
  Bus Selector2/1 -> Mux/11  "<Object_Valid[0|1]>"
  Bus Selector2/2 -> Mux/12  "<Object_Valid[0|1]>"
  Bus Selector2/3 -> Mux/13  "<Object_Valid[0|1]>"
  Bus Selector2/4 -> Mux/14  "<Object_Valid[0|1]>"
  Bus Selector2/5 -> Mux/15  "<Object_Valid[0|1]>"
  Bus Selector3/1 -> Mux1/1  "<CustomValues[]>"
  Bus Selector3/2 -> Mux1/2  "<CustomValues[]>"
  Bus Selector3/3 -> Mux1/3  "<CustomValues[]>"
  Bus Selector3/4 -> Mux1/4  "<CustomValues[]>"
  Bus Selector3/5 -> Mux1/5  "<CustomValues[]>"
  Bus Selector4/1 -> Mux1/6  "<CustomValues[]>"
  Bus Selector4/2 -> Mux1/7  "<CustomValues[]>"
  Bus Selector4/3 -> Mux1/8  "<CustomValues[]>"
  Bus Selector4/4 -> Mux1/9  "<CustomValues[]>"
  Bus Selector4/5 -> Mux1/10  "<CustomValues[]>"
  Bus Selector5/1 -> Mux1/11  "<CustomValues[]>"
  Bus Selector5/2 -> Mux1/12  "<CustomValues[]>"
  Bus Selector5/3 -> Mux1/13  "<CustomValues[]>"
  Bus Selector5/4 -> Mux1/14  "<CustomValues[]>"
  Bus Selector5/5 -> Mux1/15  "<CustomValues[]>"
  Bus Creator/1 -> Vectorized_Custom_Values/1

== system ASM_Traffic_new/Environment/Sensors/PlantModel/Object_Sensor_3D/CustomPoints/Sensor1/CustomPointsOutput/HoldSignals ==
  ResetPulse[0|1] : Inport
  CustomPoints_Signals_In[] : Inport  Port=2
  Enable : EnablePort
  Bus Selector1 : BusSelector  OutputSignals=Flag_In_Scope[0|1],Flag_Is_Occluded[0|1],ID[],Dist_CoorSys_S[m],v_CoorSys_S[m|s],v_CoorSys_S[x;y;z][m|s],a_CoorSys_S[m|s2],a_CoorSys_S[x;y;z][m|s2],Pos_CoorSys_S[x;y;z][m],Pos_CoorSys_E[x;y;z][m],Angle_Hor_CoorSys_S[deg],Angle_Ver_CoorSys_S[deg],Data_1[],Data_2[],Data_3[],Data_4[],Data_5[],Object_ID[],Object_Type[]
  CUSTOM_POINTS_SIGNALS_RESET_1 : ASM_Traffic_lib/Sensors/Custom Points/CUSTOM_POINTS_SIGNALS_RESET  ASMProperties=struct('Name','CUSTOM_POINTS_SIGNALS_RESET','Version','2.0','Library','ASM_Traffic_lib')  ASMInstanceName=custom_points_signals_reset  ASMInstanceID=1
  CustomPoints_Signals_Out[] : Outport  VectorParamsAs1DForOutWhenUnconnected=off
  wires:
  Bus Selector1/19 -> CUSTOM_POINTS_SIGNALS_RESET_1/20  "<Object_Type[]>"
  Bus Selector1/18 -> CUSTOM_POINTS_SIGNALS_RESET_1/19  "<Object_ID[]>"
  Bus Selector1/17 -> CUSTOM_POINTS_SIGNALS_RESET_1/18  "<Data_5[]>"
  Bus Selector1/16 -> CUSTOM_POINTS_SIGNALS_RESET_1/17  "<Data_4[]>"
  Bus Selector1/15 -> CUSTOM_POINTS_SIGNALS_RESET_1/16  "<Data_3[]>"
  Bus Selector1/14 -> CUSTOM_POINTS_SIGNALS_RESET_1/15  "<Data_2[]>"
  Bus Selector1/13 -> CUSTOM_POINTS_SIGNALS_RESET_1/14  "<Data_1[]>"
  Bus Selector1/12 -> CUSTOM_POINTS_SIGNALS_RESET_1/13  "<Angle_Ver_CoorSys_S[deg]>"
  Bus Selector1/11 -> CUSTOM_POINTS_SIGNALS_RESET_1/12  "<Angle_Hor_CoorSys_S[deg]>"
  Bus Selector1/10 -> CUSTOM_POINTS_SIGNALS_RESET_1/11  "<Pos_CoorSys_E[x;y;z][m]>"
  Bus Selector1/9 -> CUSTOM_POINTS_SIGNALS_RESET_1/10  "<Pos_CoorSys_S[x;y;z][m]>"
  Bus Selector1/8 -> CUSTOM_POINTS_SIGNALS_RESET_1/9  "<a_CoorSys_S[x;y;z][m|s2]>"
  Bus Selector1/7 -> CUSTOM_POINTS_SIGNALS_RESET_1/8  "<a_CoorSys_S[m|s2]>"
  Bus Selector1/6 -> CUSTOM_POINTS_SIGNALS_RESET_1/7  "<v_CoorSys_S[x;y;z][m|s]>"
  Bus Selector1/5 -> CUSTOM_POINTS_SIGNALS_RESET_1/6  "<v_CoorSys_S[m|s]>"
  Bus Selector1/4 -> CUSTOM_POINTS_SIGNALS_RESET_1/5  "<Dist_CoorSys_S[m]>"
  Bus Selector1/3 -> CUSTOM_POINTS_SIGNALS_RESET_1/4  "<ID[]>"
  Bus Selector1/2 -> CUSTOM_POINTS_SIGNALS_RESET_1/3  "<Flag_Is_Occluded[0|1]>"
  Bus Selector1/1 -> CUSTOM_POINTS_SIGNALS_RESET_1/2  "<Flag_In_Scope[0|1]>"
  CUSTOM_POINTS_SIGNALS_RESET_1/1 -> CustomPoints_Signals_Out[]/1
  ResetPulse[0|1]/1 -> CUSTOM_POINTS_SIGNALS_RESET_1/1
  CustomPoints_Signals_In[]/1 -> Bus Selector1/1

== system ASM_Traffic_new/Environment/Sensors/PlantModel/Object_Sensor_3D/CustomPoints/Sensor1/CustomPointsOutput/ResetPulse ==
  Enable[0|1] : Inport
  SensorActive[0|1] : Inport  Port=2
  Compare To Constant : simulink/Logic and Bit Operations/Compare To Constant  relop===  const=1  OutDataTypeStr=boolean
  Compare To Constant1 : simulink/Logic and Bit Operations/Compare To Constant  relop===  const=0  OutDataTypeStr=boolean
  Logical Operator1 : Logic  AllPortsSameDT=off  OutDataTypeStr=boolean
  Logical Operator2 : Logic  Operator=NAND  AllPortsSameDT=off  OutDataTypeStr=boolean
  Memory1 : UnitDelay  SampleTime=-1  HasFrameUpgradeWarning=on
  ResetPulse[0|1] : Outport  VectorParamsAs1DForOutWhenUnconnected=off
  wires:
  Enable[0|1]/1 -> Logical Operator2/2
  Compare To Constant1/1 -> Logical Operator1/2
  Compare To Constant/1 -> Logical Operator1/1
  Logical Operator1/1 -> ResetPulse[0|1]/1
  SensorActive[0|1]/1 -> Logical Operator2/1
  Logical Operator2/1 -> Memory1/1, Compare To Constant/1
  Memory1/1 -> Compare To Constant1/1

== system ASM_Traffic_new/Environment/Sensors/PlantModel/Object_Sensor_3D/CustomPoints/Sensor1/CustomPointsOutput/SignalBus ==
  CustomPoints_Signals_In[] : Inport
  Bus Creator : BusCreator  Inputs=5
  Bus Selector1 : BusSelector  OutputSignals=ID[],Object_ID[],Dist_CoorSys_S[m],Angle_Hor_CoorSys_S[deg],Pos_CoorSys_E[x;y;z][m]
  CustomPoints_Signals_Out[] : Outport  VectorParamsAs1DForOutWhenUnconnected=off
  wires:
  CustomPoints_Signals_In[]/1 -> Bus Selector1/1
  Bus Creator/1 -> CustomPoints_Signals_Out[]/1
  Bus Selector1/4 -> Bus Creator/4  "<Angle_Hor_CoorSys_S[deg]>"
  Bus Selector1/5 -> Bus Creator/5  "<Pos_CoorSys_E[x;y;z][m]>"
  Bus Selector1/2 -> Bus Creator/2  "<Object_ID[]>"
  Bus Selector1/3 -> Bus Creator/3  "<Dist_CoorSys_S[m]>"
  Bus Selector1/1 -> Bus Creator/1  "<ID[]>"

== system ASM_Traffic_new/Environment/Sensors/PlantModel/Object_Sensor_3D/CustomPoints/Sensor2/CustomPointsOutput/HoldSignals ==
  ResetPulse[0|1] : Inport
  CustomPoints_Signals_In[] : Inport  Port=2
  Enable : EnablePort
  Bus Selector1 : BusSelector  OutputSignals=Flag_In_Scope[0|1],Flag_Is_Occluded[0|1],ID[],Dist_CoorSys_S[m],v_CoorSys_S[m|s],v_CoorSys_S[x;y;z][m|s],a_CoorSys_S[m|s2],a_CoorSys_S[x;y;z][m|s2],Pos_CoorSys_S[x;y;z][m],Pos_CoorSys_E[x;y;z][m],Angle_Hor_CoorSys_S[deg],Angle_Ver_CoorSys_S[deg],Data_1[],Data_2[],Data_3[],Data_4[],Data_5[],Object_ID[],Object_Type[]
  CUSTOM_POINTS_SIGNALS_RESET_1 : ASM_Traffic_lib/Sensors/Custom Points/CUSTOM_POINTS_SIGNALS_RESET  ASMProperties=struct('Name','CUSTOM_POINTS_SIGNALS_RESET','Version','2.0','Library','ASM_Traffic_lib')  ASMInstanceName=custom_points_signals_reset  ASMInstanceID=1
  CustomPoints_Signals_Out[] : Outport  VectorParamsAs1DForOutWhenUnconnected=off
  wires:
  Bus Selector1/19 -> CUSTOM_POINTS_SIGNALS_RESET_1/20  "<Object_Type[]>"
  Bus Selector1/18 -> CUSTOM_POINTS_SIGNALS_RESET_1/19  "<Object_ID[]>"
  Bus Selector1/17 -> CUSTOM_POINTS_SIGNALS_RESET_1/18  "<Data_5[]>"
  Bus Selector1/16 -> CUSTOM_POINTS_SIGNALS_RESET_1/17  "<Data_4[]>"
  Bus Selector1/15 -> CUSTOM_POINTS_SIGNALS_RESET_1/16  "<Data_3[]>"
  Bus Selector1/14 -> CUSTOM_POINTS_SIGNALS_RESET_1/15  "<Data_2[]>"
  Bus Selector1/13 -> CUSTOM_POINTS_SIGNALS_RESET_1/14  "<Data_1[]>"
  Bus Selector1/12 -> CUSTOM_POINTS_SIGNALS_RESET_1/13  "<Angle_Ver_CoorSys_S[deg]>"
  Bus Selector1/11 -> CUSTOM_POINTS_SIGNALS_RESET_1/12  "<Angle_Hor_CoorSys_S[deg]>"
  Bus Selector1/10 -> CUSTOM_POINTS_SIGNALS_RESET_1/11  "<Pos_CoorSys_E[x;y;z][m]>"
  Bus Selector1/9 -> CUSTOM_POINTS_SIGNALS_RESET_1/10  "<Pos_CoorSys_S[x;y;z][m]>"
  Bus Selector1/8 -> CUSTOM_POINTS_SIGNALS_RESET_1/9  "<a_CoorSys_S[x;y;z][m|s2]>"
  Bus Selector1/7 -> CUSTOM_POINTS_SIGNALS_RESET_1/8  "<a_CoorSys_S[m|s2]>"
  Bus Selector1/6 -> CUSTOM_POINTS_SIGNALS_RESET_1/7  "<v_CoorSys_S[x;y;z][m|s]>"
  Bus Selector1/5 -> CUSTOM_POINTS_SIGNALS_RESET_1/6  "<v_CoorSys_S[m|s]>"
  Bus Selector1/4 -> CUSTOM_POINTS_SIGNALS_RESET_1/5  "<Dist_CoorSys_S[m]>"
  Bus Selector1/3 -> CUSTOM_POINTS_SIGNALS_RESET_1/4  "<ID[]>"
  Bus Selector1/2 -> CUSTOM_POINTS_SIGNALS_RESET_1/3  "<Flag_Is_Occluded[0|1]>"
  Bus Selector1/1 -> CUSTOM_POINTS_SIGNALS_RESET_1/2  "<Flag_In_Scope[0|1]>"
  CUSTOM_POINTS_SIGNALS_RESET_1/1 -> CustomPoints_Signals_Out[]/1
  ResetPulse[0|1]/1 -> CUSTOM_POINTS_SIGNALS_RESET_1/1
  CustomPoints_Signals_In[]/1 -> Bus Selector1/1

== system ASM_Traffic_new/Environment/Sensors/PlantModel/Object_Sensor_3D/CustomPoints/Sensor2/CustomPointsOutput/ResetPulse ==
  Enable[0|1] : Inport
  SensorActive[0|1] : Inport  Port=2
  Compare To Constant : simulink/Logic and Bit Operations/Compare To Constant  relop===  const=1  OutDataTypeStr=boolean
  Compare To Constant1 : simulink/Logic and Bit Operations/Compare To Constant  relop===  const=0  OutDataTypeStr=boolean
  Logical Operator1 : Logic  AllPortsSameDT=off  OutDataTypeStr=boolean
  Logical Operator2 : Logic  Operator=NAND  AllPortsSameDT=off  OutDataTypeStr=boolean
  Memory1 : UnitDelay  SampleTime=-1  HasFrameUpgradeWarning=on
  ResetPulse[0|1] : Outport  VectorParamsAs1DForOutWhenUnconnected=off
  wires:
  Enable[0|1]/1 -> Logical Operator2/2
  Compare To Constant1/1 -> Logical Operator1/2
  Compare To Constant/1 -> Logical Operator1/1
  Logical Operator1/1 -> ResetPulse[0|1]/1
  SensorActive[0|1]/1 -> Logical Operator2/1
  Logical Operator2/1 -> Memory1/1, Compare To Constant/1
  Memory1/1 -> Compare To Constant1/1

== system ASM_Traffic_new/Environment/Sensors/PlantModel/Object_Sensor_3D/CustomPoints/Sensor2/CustomPointsOutput/SignalBus ==
  CustomPoints_Signals_In[] : Inport
  Bus Creator : BusCreator  Inputs=5
  Bus Selector1 : BusSelector  OutputSignals=ID[],Object_ID[],Dist_CoorSys_S[m],Angle_Hor_CoorSys_S[deg],Pos_CoorSys_E[x;y;z][m]
  CustomPoints_Signals_Out[] : Outport  VectorParamsAs1DForOutWhenUnconnected=off
  wires:
  CustomPoints_Signals_In[]/1 -> Bus Selector1/1
  Bus Creator/1 -> CustomPoints_Signals_Out[]/1
  Bus Selector1/4 -> Bus Creator/4  "<Angle_Hor_CoorSys_S[deg]>"
  Bus Selector1/5 -> Bus Creator/5  "<Pos_CoorSys_E[x;y;z][m]>"
  Bus Selector1/2 -> Bus Creator/2  "<Object_ID[]>"
  Bus Selector1/3 -> Bus Creator/3  "<Dist_CoorSys_S[m]>"
  Bus Selector1/1 -> Bus Creator/1  "<ID[]>"

== system ASM_Traffic_new/Environment/Sensors/PlantModel/Object_Sensor_3D/CustomPoints/Sensor3/CustomPointsOutput/HoldSignals ==
  ResetPulse[0|1] : Inport
  CustomPoints_Signals_In[] : Inport  Port=2
  Enable : EnablePort
  Bus Selector1 : BusSelector  OutputSignals=Flag_In_Scope[0|1],Flag_Is_Occluded[0|1],ID[],Dist_CoorSys_S[m],v_CoorSys_S[m|s],v_CoorSys_S[x;y;z][m|s],a_CoorSys_S[m|s2],a_CoorSys_S[x;y;z][m|s2],Pos_CoorSys_S[x;y;z][m],Pos_CoorSys_E[x;y;z][m],Angle_Hor_CoorSys_S[deg],Angle_Ver_CoorSys_S[deg],Data_1[],Data_2[],Data_3[],Data_4[],Data_5[],Object_ID[],Object_Type[]
  CUSTOM_POINTS_SIGNALS_RESET_1 : ASM_Traffic_lib/Sensors/Custom Points/CUSTOM_POINTS_SIGNALS_RESET  ASMProperties=struct('Name','CUSTOM_POINTS_SIGNALS_RESET','Version','2.0','Library','ASM_Traffic_lib')  ASMInstanceName=custom_points_signals_reset  ASMInstanceID=1
  CustomPoints_Signals_Out[] : Outport  VectorParamsAs1DForOutWhenUnconnected=off
  wires:
  Bus Selector1/19 -> CUSTOM_POINTS_SIGNALS_RESET_1/20  "<Object_Type[]>"
  Bus Selector1/18 -> CUSTOM_POINTS_SIGNALS_RESET_1/19  "<Object_ID[]>"
  Bus Selector1/17 -> CUSTOM_POINTS_SIGNALS_RESET_1/18  "<Data_5[]>"
  Bus Selector1/16 -> CUSTOM_POINTS_SIGNALS_RESET_1/17  "<Data_4[]>"
  Bus Selector1/15 -> CUSTOM_POINTS_SIGNALS_RESET_1/16  "<Data_3[]>"
  Bus Selector1/14 -> CUSTOM_POINTS_SIGNALS_RESET_1/15  "<Data_2[]>"
  Bus Selector1/13 -> CUSTOM_POINTS_SIGNALS_RESET_1/14  "<Data_1[]>"
  Bus Selector1/12 -> CUSTOM_POINTS_SIGNALS_RESET_1/13  "<Angle_Ver_CoorSys_S[deg]>"
  Bus Selector1/11 -> CUSTOM_POINTS_SIGNALS_RESET_1/12  "<Angle_Hor_CoorSys_S[deg]>"
  Bus Selector1/10 -> CUSTOM_POINTS_SIGNALS_RESET_1/11  "<Pos_CoorSys_E[x;y;z][m]>"
  Bus Selector1/9 -> CUSTOM_POINTS_SIGNALS_RESET_1/10  "<Pos_CoorSys_S[x;y;z][m]>"
  Bus Selector1/8 -> CUSTOM_POINTS_SIGNALS_RESET_1/9  "<a_CoorSys_S[x;y;z][m|s2]>"
  Bus Selector1/7 -> CUSTOM_POINTS_SIGNALS_RESET_1/8  "<a_CoorSys_S[m|s2]>"
  Bus Selector1/6 -> CUSTOM_POINTS_SIGNALS_RESET_1/7  "<v_CoorSys_S[x;y;z][m|s]>"
  Bus Selector1/5 -> CUSTOM_POINTS_SIGNALS_RESET_1/6  "<v_CoorSys_S[m|s]>"
  Bus Selector1/4 -> CUSTOM_POINTS_SIGNALS_RESET_1/5  "<Dist_CoorSys_S[m]>"
  Bus Selector1/3 -> CUSTOM_POINTS_SIGNALS_RESET_1/4  "<ID[]>"
  Bus Selector1/2 -> CUSTOM_POINTS_SIGNALS_RESET_1/3  "<Flag_Is_Occluded[0|1]>"
  Bus Selector1/1 -> CUSTOM_POINTS_SIGNALS_RESET_1/2  "<Flag_In_Scope[0|1]>"
  CUSTOM_POINTS_SIGNALS_RESET_1/1 -> CustomPoints_Signals_Out[]/1
  ResetPulse[0|1]/1 -> CUSTOM_POINTS_SIGNALS_RESET_1/1
  CustomPoints_Signals_In[]/1 -> Bus Selector1/1

== system ASM_Traffic_new/Environment/Sensors/PlantModel/Object_Sensor_3D/CustomPoints/Sensor3/CustomPointsOutput/ResetPulse1 ==
  Enable[0|1] : Inport
  SensorActive[0|1] : Inport  Port=2
  Compare To Constant : simulink/Logic and Bit Operations/Compare To Constant  relop===  const=1  OutDataTypeStr=boolean
  Compare To Constant1 : simulink/Logic and Bit Operations/Compare To Constant  relop===  const=0  OutDataTypeStr=boolean
  Logical Operator1 : Logic  AllPortsSameDT=off  OutDataTypeStr=boolean
  Logical Operator2 : Logic  Operator=NAND  AllPortsSameDT=off  OutDataTypeStr=boolean
  Memory1 : UnitDelay  SampleTime=-1  HasFrameUpgradeWarning=on
  ResetPulse[0|1] : Outport  VectorParamsAs1DForOutWhenUnconnected=off
  wires:
  Enable[0|1]/1 -> Logical Operator2/2
  Compare To Constant1/1 -> Logical Operator1/2
  Compare To Constant/1 -> Logical Operator1/1
  Logical Operator1/1 -> ResetPulse[0|1]/1
  SensorActive[0|1]/1 -> Logical Operator2/1
  Logical Operator2/1 -> Memory1/1, Compare To Constant/1
  Memory1/1 -> Compare To Constant1/1

== system ASM_Traffic_new/Environment/Sensors/PlantModel/Object_Sensor_3D/CustomPoints/Sensor3/CustomPointsOutput/SignalBus ==
  CustomPoints_Signals_In[] : Inport
  Bus Creator : BusCreator  Inputs=5
  Bus Selector1 : BusSelector  OutputSignals=ID[],Object_ID[],Dist_CoorSys_S[m],Angle_Hor_CoorSys_S[deg],Pos_CoorSys_E[x;y;z][m]
  CustomPoints_Signals_Out[] : Outport  VectorParamsAs1DForOutWhenUnconnected=off
  wires:
  CustomPoints_Signals_In[]/1 -> Bus Selector1/1
  Bus Creator/1 -> CustomPoints_Signals_Out[]/1
  Bus Selector1/4 -> Bus Creator/4  "<Angle_Hor_CoorSys_S[deg]>"
  Bus Selector1/5 -> Bus Creator/5  "<Pos_CoorSys_E[x;y;z][m]>"
  Bus Selector1/2 -> Bus Creator/2  "<Object_ID[]>"
  Bus Selector1/3 -> Bus Creator/3  "<Dist_CoorSys_S[m]>"
  Bus Selector1/1 -> Bus Creator/1  "<ID[]>"

== system ASM_Traffic_new/Environment/Sensors/PlantModel/Object_Sensor_3D/ObjectData/BoundingBoxData_CoorSys_E/BoundingBoxData_CoorSys_E/GetFellowPositionVector ==
  <FellowPositions> : Inport
  Bus Selector11 : BusSelector  OutputSignals=Pos_Fellows_MainPnt_CoorSys_E[x;y;z][m].Pos_x_Fellows[m],Pos_Fellows_MainPnt_CoorSys_E[x;y;z][m].Pos_y_Fellows[m],Pos_Fellows_MainPnt_CoorSys_E[x;y;z][m].Pos_z_Fellows[m],Angle_Fellows[x;y;z][deg].Angle_Roll_Fellows[deg],Angle_Fellows[x;y;z][deg].Angle_Pitch_Fellows[deg],Angle_Fellows[x;y;z][deg].Angle_Yaw_Fellows[deg]
  Mux1 : Mux  Inputs=3
  Mux2 : Mux  Inputs=3
  Pos_Fellows_MainPnt_CoorSys_E[x;y;z][m] : Outport  VectorParamsAs1DForOutWhenUnconnected=off
  Angle_Fellows[deg] : Outport  Port=2  VectorParamsAs1DForOutWhenUnconnected=off
  wires:
  Mux2/1 -> Pos_Fellows_MainPnt_CoorSys_E[x;y;z][m]/1  "Pos_Fellows_MainPnt_CoorSys_E[x;y;z][m]"
  Mux1/1 -> Angle_Fellows[deg]/1  "Pos_Fellows_MainPnt_CoorSys_E_vec"
  Bus Selector11/4 -> Mux1/1  "<Angle_Roll_Fellows[deg]>"
  Bus Selector11/1 -> Mux2/1  "<Pos_x_Fellows[m]>"
  Bus Selector11/2 -> Mux2/2  "<Pos_y_Fellows[m]>"
  Bus Selector11/6 -> Mux1/3  "<Angle_Yaw_Fellows[deg]>"
  Bus Selector11/5 -> Mux1/2  "<Angle_Pitch_Fellows[deg]>"
  <FellowPositions>/1 -> Bus Selector11/1
  Bus Selector11/3 -> Mux2/3  "<Pos_z_Fellows[m]>"
